simulink model "LQRI_linear_sim"  (R2026a)
settings: Solver=VariableStepAuto
InitFcn:
  | actuator = actuator_params_nominal();
  | [Gact, info] = build_nominal_actuator(actuator);
  | 
  | % Parametri del robot
  | p = sea_params_nominal();
  | Simulink.Bus.createObject(p);
  | 
  | % Equilibrio desiderato
  | qbar = [pi/2; 0];
  | 
  | % Calcolo stato e coppia di equilibrio
  | [xbar, taubar, info] = sea_static_equilibrium(qbar, p);
undefined symbols (not defined in the file): A, B, C, Ki, Kx, L
settings Model: Creator=rebec  LastModifiedBy=rebec

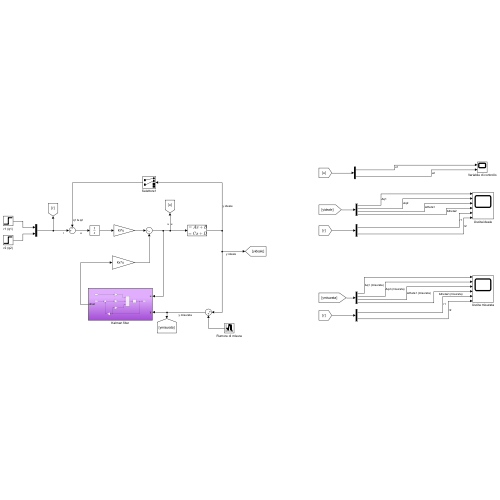
[thumbnail: Simulink's stored preview of the top-level diagram]
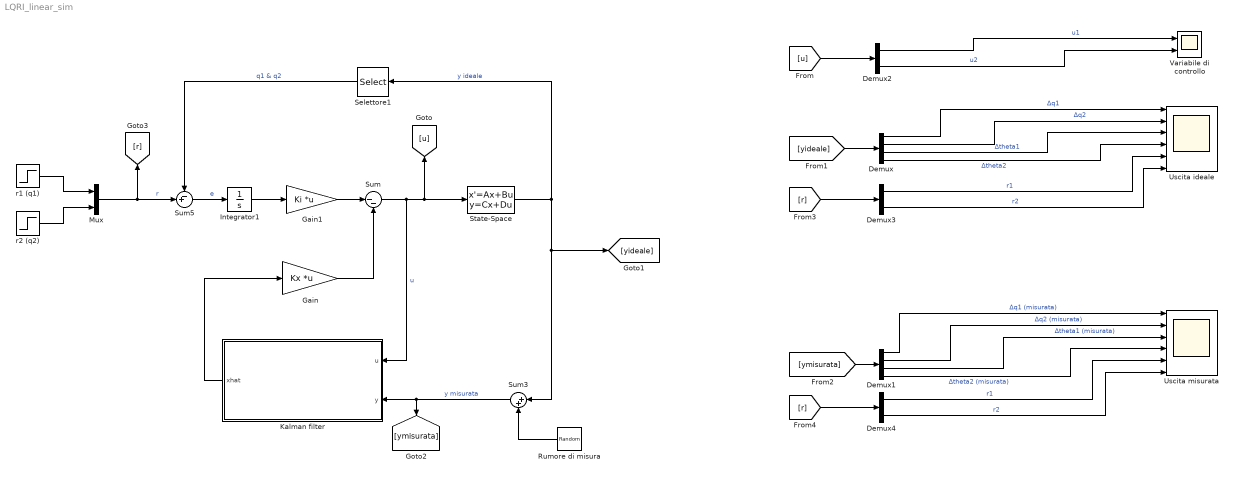
== system LQRI_linear_sim ==
  Demux : Demux
  Demux1 : Demux
  Demux2 : Demux  Outputs=2
  Demux3 : Demux  Outputs=2
  Demux4 : Demux  Outputs=2
  Gain : Gain  Gain=Kx  Multiplication=Matrix(K*u)
  Gain1 : Gain  Gain=Ki  Multiplication=Matrix(K*u)
  Integrator1 : Integrator
  Kalman filter : Subsystem
  Mux : Mux  Inputs=2
  Rumore di misura : RandomNumber  Variance=(0.05*pi/180)^2  Seed=20260826  SampleTime=0.002
  Selettore1 : Selector  InputPortWidth=4  IndexOptions=Index vector (dialog)  Indices=[1 2]  OutputSizes=1
  State-Space : StateSpace  A=A  B=B  C=C  D=zeros(4,2);  InitialCondition=0
  Sum : Sum  Inputs=|--
  Sum3 : Sum  Inputs=|++
  Sum5 : Sum  Inputs=-+|
  Uscita ideale : Scope  NumInputPorts=6
      settings: Title=y (uscita ideale)  ActiveDisplayYMinimum=-0.25184604683047779  ActiveDisplayYMaximum=0.2822060996012532
  Uscita misurata : Scope  NumInputPorts=6
      settings: Title=y (uscita ideale)  ActiveDisplayYMinimum=-0.10972330467546007  ActiveDisplayYMaximum=0.17651509397452056
  Variabile di controllo : Scope  NumInputPorts=2
      settings: ActiveDisplayYMinimum=-2.6959450601265313  ActiveDisplayYMaximum=5.9059369724787079  DataLoggingVariableName=ScopeData2
  r1 (q1) : Step  FinalValue=5*pi/180  SampleTime=0
  r2 (q2) : Step  FinalValue=0  SampleTime=0
  wires:
  Gain1/1 -> Sum/1
  Demux/1 -> Uscita ideale/1  "Δq1"
  [r] -> Demux4/1
  Demux/2 -> Uscita ideale/2  "Δq2"
  Mux/1 -> [r], Sum5/2  "r"
  [u] -> Demux2/1
  [yideale] -> Demux/1
  Demux1/3 -> Uscita misurata/3  "Δtheta1 (misurata)"
  Sum3/1 -> Kalman filter/2(y), [ymisurata]  "y misurata"
  Demux4/2 -> Uscita misurata/6  "r2"
  Demux4/1 -> Uscita misurata/5  "r1"
  Sum/1 -> Kalman filter/1(u), [u], State-Space/1  "u"
  Rumore di misura/1 -> Sum3/2
  Demux2/1 -> Variabile di controllo/1  "u1"
  [ymisurata] -> Demux1/1
  Demux/3 -> Uscita ideale/3  "Δtheta1"
  Integrator1/1 -> Gain1/1
  r2 (q2)/1 -> Mux/2
  Gain/1 -> Sum/2
  Demux/4 -> Uscita ideale/4  "Δtheta2"
  Selettore1/1 -> Sum5/1  "q1 & q2"
  Demux1/2 -> Uscita misurata/2  "Δq2 (misurata)"
  Demux2/2 -> Variabile di controllo/2  "u2"
  Demux3/1 -> Uscita ideale/5  "r1"
  Demux1/1 -> Uscita misurata/1  "Δq1 (misurata)"
  Sum5/1 -> Integrator1/1  "e"
  r1 (q1)/1 -> Mux/1
  Demux3/2 -> Uscita ideale/6  "r2"
  [r] -> Demux3/1
  Demux1/4 -> Uscita misurata/4  "Δtheta2 (misurata)"
  Kalman filter/1(xhat) -> Gain/1
  State-Space/1 -> Selettore1/1, [yideale], Sum3/1  "y ideale"

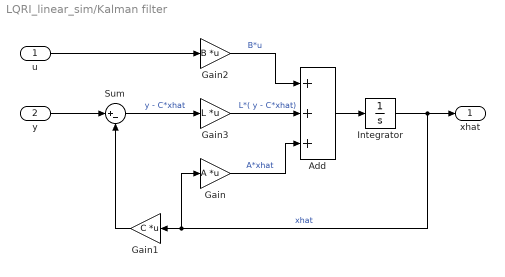
== system LQRI_linear_sim/Kalman filter ==
  u : Inport
  y : Inport  Port=2
  Add : Sum  Inputs=+++
  Gain : Gain  Gain=A  Multiplication=Matrix(K*u)
  Gain1 : Gain  Gain=C  Multiplication=Matrix(K*u)
  Gain2 : Gain  Gain=B  Multiplication=Matrix(K*u)
  Gain3 : Gain  Gain=L  Multiplication=Matrix(K*u)
  Integrator : Integrator
  Sum : Sum  Inputs=|+-
  xhat : Outport
  wires:
  u/1 -> Gain2/1
  y/1 -> Sum/1
  Gain1/1 -> Sum/2
  Sum/1 -> Gain3/1  "y - C*xhat"
  Gain3/1 -> Add/2  "L*( y - C*xhat)"
  Gain2/1 -> Add/1  "B*u"
  Gain/1 -> Add/3  "A*xhat"
  Add/1 -> Integrator/1
  Integrator/1 -> Gain/1, Gain1/1, xhat/1  "xhat"
